simulink model "kay1024_freq_16ch_test"  (R2021b)
settings: Solver=VariableStepAuto  StartTime=0.0  StopTime=10.0  RelTol=1e-3
undefined symbols (not defined in the file): i
libraries: hdlBasic x1194, dspsrcs4 x16, vmcUtilities x1
(part 2 of 14)

== system kay1024_freq_16ch_test/Subsystem/Subsystem16/Subsystem7 ==
  In1 : Inport
  In2 : Inport  Port=2
  In3 : Inport  Port=3
  In4 : Inport  Port=4
  CORDIC ATAN : Subsystem  mask(Xilinx CORDIC ATAN){stages=15, pe_nbits=30, pe_binpt=18, pipeline_x=ones(1,15), prev_stages=15, pipeline=[1  1  1  1  1  1  1  1  1  1  1  1  1  1  1]}
      mask prompts: stages "Number of Processing Elements (integer value starting from 1)"; pe_nbits "X, Y Data Width"; pe_binpt "X, Y Binary Point Position"; pipeline_x "Latency for each Processing Element [1 0 0 1]"; prev_stages "Previous Number of Stages"; pipeline "Previous Pipeline Values"
      mask help: A parallel implementation, circular vectoring mode CORDIC processor for performing rectangular-to-polar conversion. The number of iteration stages (and resultant output accuracy) and the processor arithmetic precision are controlled by the mask customization.
      mask init: same as kay1024_freq_16ch_test/Subsystem/Subsystem16/Subsystem/CORDIC ATAN
      settings: CopyFcn=set_param(gcb, 'MaskSelfModifiable', 'on', 'LinkStatus', 'none');
      mask Help: eval('');xlDoc('-book','sysgen','-topic','CORDIC_ATAN');
      mask Display:
      | patch([0 iWidth iWidth 0],[0 0 iHeight iHeight] , bg);
      | patch(logoX,logoY , fg);
      | text(iCx-6,iCy,'z');
      | text(iCx,iCy+4,str);
      | port_label('input',1,'x');
      | port_label('input',2,'y');
      | port_label('output',1,'mag');
      | port_label('output',2,'atan');
      | plot([0 0 iWidth iWidth 0], [0 iHeight iHeight 0 0]);
  im0*im1 : hdlBasic/Mult  precision=Full  arith_type="Signed  (2's comp)"  n_bits=16  bin_pt=14  quantization=Truncate  overflow=Wrap  en=off  latency=3  use_behavioral_HDL=off  opt=Speed  use_embedded=on  optimum_pipeline=off  pipeline=on  use_rpm=on  placement_style=Triangular  XmcBlockStatus=1  maskContainerNames=group1  block_type=mult  block_config=sysgen:Mult_config  block_width=598  block_height=876
  re0*im1 : hdlBasic/Mult  precision=Full  arith_type="Signed  (2's comp)"  n_bits=16  bin_pt=14  quantization=Truncate  overflow=Wrap  en=off  latency=3  use_behavioral_HDL=off  opt=Speed  use_embedded=on  optimum_pipeline=off  pipeline=on  use_rpm=on  placement_style=Triangular  XmcBlockStatus=1  maskContainerNames=group1  block_type=mult  block_config=sysgen:Mult_config  block_width=598  block_height=876
  re0*im1-re1*im0 : hdlBasic/AddSub  mode=Subtraction  use_carryin=off  use_carryout=off  en=off  latency=1  precision=Full  arith_type=Unsigned  n_bits=16  bin_pt=14  quantization=Truncate  overflow=Wrap  use_behavioral_HDL=off  hw_selection=Fabric  pipelined=off  XmcBlockStatus=1  maskContainerNames=tabcontainer1  block_type=addsub  block_config=sysgen:Addsub_config
  re0*re1 : hdlBasic/Mult  precision=Full  arith_type="Signed  (2's comp)"  n_bits=16  bin_pt=14  quantization=Truncate  overflow=Wrap  en=off  latency=3  use_behavioral_HDL=off  opt=Speed  use_embedded=on  optimum_pipeline=off  pipeline=on  use_rpm=on  placement_style=Triangular  XmcBlockStatus=1  maskContainerNames=group1  block_type=mult  block_config=sysgen:Mult_config  block_width=598  block_height=876
  re0*re1+im0*im1 : hdlBasic/AddSub  mode=Addition  use_carryin=off  use_carryout=off  en=off  latency=1  precision=Full  arith_type=Unsigned  n_bits=16  bin_pt=14  quantization=Truncate  overflow=Wrap  use_behavioral_HDL=off  hw_selection=Fabric  pipelined=off  XmcBlockStatus=1  maskContainerNames=tabcontainer1  block_type=addsub  block_config=sysgen:Addsub_config
  re1*im0 : hdlBasic/Mult  precision=Full  arith_type="Signed  (2's comp)"  n_bits=16  bin_pt=14  quantization=Truncate  overflow=Wrap  en=off  latency=3  use_behavioral_HDL=off  opt=Speed  use_embedded=on  optimum_pipeline=off  pipeline=on  use_rpm=on  placement_style=Triangular  XmcBlockStatus=1  maskContainerNames=group1  block_type=mult  block_config=sysgen:Mult_config  block_width=598  block_height=876
  Z : Outport
  wires:
  In3/1 -> re1*im0/2, im0*im1/1
  re0*im1-re1*im0/1 -> CORDIC ATAN/2(y)
  In2/1 -> re0*re1/2, re1*im0/1
  In4/1 -> re0*im1/2, im0*im1/2
  re0*im1/1 -> re0*im1-re1*im0/1
  In1/1 -> re0*im1/1, re0*re1/1
  re0*re1/1 -> re0*re1+im0*im1/1
  im0*im1/1 -> re0*re1+im0*im1/2
  re0*re1+im0*im1/1 -> CORDIC ATAN/1(x)
  re1*im0/1 -> re0*im1-re1*im0/2
  CORDIC ATAN/2(Z) -> Z/1

== system kay1024_freq_16ch_test/Subsystem/Subsystem16/Subsystem/CORDIC ATAN ==
  note: The CORDIC algorithm is implemented in 3 steps.
      |
      | Step 1: Coarse Angle Rotation.  The algorithm converges only for angles between -pi/2 and pi/2, so if x < zero, the input vector is reflected
      | to the 1st or 3rd quadrant by making the x-coordinate non-negative.
      |
      | Step 2: Fine Angle Rotation.  For rectangular-to-polar conversion, the resulting vector is rotated through progressively smaller angles, such that y goes
      | to zero. In the i-th stage, the angular rotation is by either +/- atan(1/2^i), depending on whether or not its input y is less than or greater than zero.
      |
      | Step 3: Angle Correction. If there was a reflection applied in Step 1, this step applies the appropriate angle correction by subtracting it from +/- pi.
  x : Inport
  y : Inport  Port=2
  CORDIC Pipe Balance : hdlBasic/Delay  rst=off  en=off  latency=sum(pipeline)  reg_retiming=off  XmcBlockStatus=1  maskContainerNames=group1  block_type=delay  block_config=sysgen:Delay_config
  CORDIC Pipe Balance1 : hdlBasic/Delay  rst=off  en=off  latency=sum(pipeline)+1  reg_retiming=off  XmcBlockStatus=1  maskContainerNames=group1  block_type=delay  block_config=sysgen:Delay_config
  CORDIC Pipe Balance2 : hdlBasic/Delay  rst=off  en=off  latency=1  reg_retiming=off  XmcBlockStatus=1  maskContainerNames=group1  block_type=delay  block_config=sysgen:Delay_config
  CORDIC Fine Angle PE : Subsystem  mask(CORDIC parallel PE){}
      mask init:
      | [bg,fg] = xlcmap('XBlock',0);
      | iPos = get_param(gcb,'Position');
      | iWidth=iPos(3)-iPos(1); iHeight=iPos(4)-iPos(2);
      | iCx=iWidth/2;
      | iCy=iHeight/2;
      | [logoX, logoY] = xlogo(iPos);
      mask Display:
      | patch([0 iWidth iWidth 0],[0 0 iHeight iHeight] , bg);
      | patch(logoX,logoY , fg);
      | port_label('input',1,'x');
      | port_label('input',2,'y');
      | port_label('input',3,'z');
      | port_label('output',1,'X');
      | port_label('output',2,'Z');
      | plot([0 0 iWidth iWidth 0], [0 iHeight iHeight 0 0]);
  Constant : hdlBasic/Constant  const=0  gui_display_data_type=Fixed-point  arith_type=Signed (2's comp)  n_bits=pe_nbits  bin_pt=pe_binpt  preci_type=Single  exp_width=8  frac_width=24  explicit_period=off  period=1  XmcBlockStatus=1  maskContainerNames=tabcontainer1  block_type=constant  block_config=sysgen:Constant_config
  Quadrant Correct : Subsystem
      mask init:
      | [bg,fg] = xlcmap('XBlock',0);
      | iPos = get_param(gcb,'Position');
      | iWidth=iPos(3)-iPos(1); iHeight=iPos(4)-iPos(2);
      | iCx=iWidth/2;
      | iCy=iHeight/2;
      | [logoX, logoY] = xlogo(iPos);
      mask Display:
      | patch([0 iWidth iWidth 0],[0 0 iHeight iHeight] , bg);
      | patch(logoX,logoY , fg);
      | port_label('input',1,'Z in');
      | port_label('input',2,'sgn(y)');
      | port_label('input',3,'sgn(x)');
      | port_label('output',1,'Z');
      | plot([0 0 iWidth iWidth 0], [0 iHeight iHeight 0 0]);
  Quadrant Map : Subsystem
      mask init:
      | [bg,fg] = xlcmap('XBlock',0);
      | iPos = get_param(gcb,'Position');
      | iWidth=iPos(3)-iPos(1); iHeight=iPos(4)-iPos(2);
      | iCx=iWidth/2;
      | iCy=iHeight/2;
      | [logoX, logoY] = xlogo(iPos);
      mask Display:
      | patch([0 iWidth iWidth 0],[0 0 iHeight iHeight] , bg);
      | patch(logoX,logoY , fg);
      | port_label('input',1,'x');
      | port_label('input',2,'y');
      | port_label('output',1,'X');
      | port_label('output',2,'Y');
      | port_label('output',3,'sgn(y)');
      | port_label('output',4,'sgn(x)');
      | plot([0 0 iWidth iWidth 0], [0 iHeight iHeight 0 0]);
  X : Outport
  Z : Outport  Port=2
  wires:
  CORDIC Pipe Balance2/1 -> X/1
  CORDIC Fine Angle PE/1(X) -> CORDIC Pipe Balance2/1
  Quadrant Correct/1(Z) -> Z/1
  CORDIC Fine Angle PE/2(Z) -> Quadrant Correct/1(Z IN)
  CORDIC Pipe Balance1/1 -> Quadrant Correct/3(Z MUX SEL)
  CORDIC Pipe Balance/1 -> Quadrant Correct/2(PI_ addsub)
  Quadrant Map/4(sign(x)) -> CORDIC Pipe Balance1/1
  Quadrant Map/3(sign(y)) -> CORDIC Pipe Balance/1
  y/1 -> Quadrant Map/2(y)
  x/1 -> Quadrant Map/1(x)
  Quadrant Map/2(Y) -> CORDIC Fine Angle PE/2(y)
  Quadrant Map/1(X) -> CORDIC Fine Angle PE/1(x)
  Constant/1 -> CORDIC Fine Angle PE/3(z)

== system kay1024_freq_16ch_test/Subsystem/Subsystem16/Subsystem1/CORDIC ATAN ==
  note: The CORDIC algorithm is implemented in 3 steps.
      |
      | Step 1: Coarse Angle Rotation.  The algorithm converges only for angles between -pi/2 and pi/2, so if x < zero, the input vector is reflected
      | to the 1st or 3rd quadrant by making the x-coordinate non-negative.
      |
      | Step 2: Fine Angle Rotation.  For rectangular-to-polar conversion, the resulting vector is rotated through progressively smaller angles, such that y goes
      | to zero. In the i-th stage, the angular rotation is by either +/- atan(1/2^i), depending on whether or not its input y is less than or greater than zero.
      |
      | Step 3: Angle Correction. If there was a reflection applied in Step 1, this step applies the appropriate angle correction by subtracting it from +/- pi.
  x : Inport
  y : Inport  Port=2
  CORDIC Pipe Balance : hdlBasic/Delay  rst=off  en=off  latency=sum(pipeline)  reg_retiming=off  XmcBlockStatus=1  maskContainerNames=group1  block_type=delay  block_config=sysgen:Delay_config
  CORDIC Pipe Balance1 : hdlBasic/Delay  rst=off  en=off  latency=sum(pipeline)+1  reg_retiming=off  XmcBlockStatus=1  maskContainerNames=group1  block_type=delay  block_config=sysgen:Delay_config
  CORDIC Pipe Balance2 : hdlBasic/Delay  rst=off  en=off  latency=1  reg_retiming=off  XmcBlockStatus=1  maskContainerNames=group1  block_type=delay  block_config=sysgen:Delay_config
  CORDIC Fine Angle PE : Subsystem  mask(CORDIC parallel PE){}
      mask init:
      | [bg,fg] = xlcmap('XBlock',0);
      | iPos = get_param(gcb,'Position');
      | iWidth=iPos(3)-iPos(1); iHeight=iPos(4)-iPos(2);
      | iCx=iWidth/2;
      | iCy=iHeight/2;
      | [logoX, logoY] = xlogo(iPos);
      mask Display:
      | patch([0 iWidth iWidth 0],[0 0 iHeight iHeight] , bg);
      | patch(logoX,logoY , fg);
      | port_label('input',1,'x');
      | port_label('input',2,'y');
      | port_label('input',3,'z');
      | port_label('output',1,'X');
      | port_label('output',2,'Z');
      | plot([0 0 iWidth iWidth 0], [0 iHeight iHeight 0 0]);
  Constant : hdlBasic/Constant  const=0  gui_display_data_type=Fixed-point  arith_type=Signed (2's comp)  n_bits=pe_nbits  bin_pt=pe_binpt  preci_type=Single  exp_width=8  frac_width=24  explicit_period=off  period=1  XmcBlockStatus=1  maskContainerNames=tabcontainer1  block_type=constant  block_config=sysgen:Constant_config
  Quadrant Correct : Subsystem
      mask init:
      | [bg,fg] = xlcmap('XBlock',0);
      | iPos = get_param(gcb,'Position');
      | iWidth=iPos(3)-iPos(1); iHeight=iPos(4)-iPos(2);
      | iCx=iWidth/2;
      | iCy=iHeight/2;
      | [logoX, logoY] = xlogo(iPos);
      mask Display:
      | patch([0 iWidth iWidth 0],[0 0 iHeight iHeight] , bg);
      | patch(logoX,logoY , fg);
      | port_label('input',1,'Z in');
      | port_label('input',2,'sgn(y)');
      | port_label('input',3,'sgn(x)');
      | port_label('output',1,'Z');
      | plot([0 0 iWidth iWidth 0], [0 iHeight iHeight 0 0]);
  Quadrant Map : Subsystem
      mask init:
      | [bg,fg] = xlcmap('XBlock',0);
      | iPos = get_param(gcb,'Position');
      | iWidth=iPos(3)-iPos(1); iHeight=iPos(4)-iPos(2);
      | iCx=iWidth/2;
      | iCy=iHeight/2;
      | [logoX, logoY] = xlogo(iPos);
      mask Display:
      | patch([0 iWidth iWidth 0],[0 0 iHeight iHeight] , bg);
      | patch(logoX,logoY , fg);
      | port_label('input',1,'x');
      | port_label('input',2,'y');
      | port_label('output',1,'X');
      | port_label('output',2,'Y');
      | port_label('output',3,'sgn(y)');
      | port_label('output',4,'sgn(x)');
      | plot([0 0 iWidth iWidth 0], [0 iHeight iHeight 0 0]);
  X : Outport
  Z : Outport  Port=2
  wires:
  CORDIC Pipe Balance2/1 -> X/1
  CORDIC Fine Angle PE/1(X) -> CORDIC Pipe Balance2/1
  Quadrant Correct/1(Z) -> Z/1
  CORDIC Fine Angle PE/2(Z) -> Quadrant Correct/1(Z IN)
  CORDIC Pipe Balance1/1 -> Quadrant Correct/3(Z MUX SEL)
  CORDIC Pipe Balance/1 -> Quadrant Correct/2(PI_ addsub)
  Quadrant Map/4(sign(x)) -> CORDIC Pipe Balance1/1
  Quadrant Map/3(sign(y)) -> CORDIC Pipe Balance/1
  y/1 -> Quadrant Map/2(y)
  x/1 -> Quadrant Map/1(x)
  Quadrant Map/2(Y) -> CORDIC Fine Angle PE/2(y)
  Quadrant Map/1(X) -> CORDIC Fine Angle PE/1(x)
  Constant/1 -> CORDIC Fine Angle PE/3(z)

== system kay1024_freq_16ch_test/Subsystem/Subsystem16/Subsystem2/CORDIC ATAN ==
  note: The CORDIC algorithm is implemented in 3 steps.
      |
      | Step 1: Coarse Angle Rotation.  The algorithm converges only for angles between -pi/2 and pi/2, so if x < zero, the input vector is reflected
      | to the 1st or 3rd quadrant by making the x-coordinate non-negative.
      |
      | Step 2: Fine Angle Rotation.  For rectangular-to-polar conversion, the resulting vector is rotated through progressively smaller angles, such that y goes
      | to zero. In the i-th stage, the angular rotation is by either +/- atan(1/2^i), depending on whether or not its input y is less than or greater than zero.
      |
      | Step 3: Angle Correction. If there was a reflection applied in Step 1, this step applies the appropriate angle correction by subtracting it from +/- pi.
  x : Inport
  y : Inport  Port=2
  CORDIC Pipe Balance : hdlBasic/Delay  rst=off  en=off  latency=sum(pipeline)  reg_retiming=off  XmcBlockStatus=1  maskContainerNames=group1  block_type=delay  block_config=sysgen:Delay_config
  CORDIC Pipe Balance1 : hdlBasic/Delay  rst=off  en=off  latency=sum(pipeline)+1  reg_retiming=off  XmcBlockStatus=1  maskContainerNames=group1  block_type=delay  block_config=sysgen:Delay_config
  CORDIC Pipe Balance2 : hdlBasic/Delay  rst=off  en=off  latency=1  reg_retiming=off  XmcBlockStatus=1  maskContainerNames=group1  block_type=delay  block_config=sysgen:Delay_config
  CORDIC Fine Angle PE : Subsystem  mask(CORDIC parallel PE){}
      mask init:
      | [bg,fg] = xlcmap('XBlock',0);
      | iPos = get_param(gcb,'Position');
      | iWidth=iPos(3)-iPos(1); iHeight=iPos(4)-iPos(2);
      | iCx=iWidth/2;
      | iCy=iHeight/2;
      | [logoX, logoY] = xlogo(iPos);
      mask Display:
      | patch([0 iWidth iWidth 0],[0 0 iHeight iHeight] , bg);
      | patch(logoX,logoY , fg);
      | port_label('input',1,'x');
      | port_label('input',2,'y');
      | port_label('input',3,'z');
      | port_label('output',1,'X');
      | port_label('output',2,'Z');
      | plot([0 0 iWidth iWidth 0], [0 iHeight iHeight 0 0]);
  Constant : hdlBasic/Constant  const=0  gui_display_data_type=Fixed-point  arith_type=Signed (2's comp)  n_bits=pe_nbits  bin_pt=pe_binpt  preci_type=Single  exp_width=8  frac_width=24  explicit_period=off  period=1  XmcBlockStatus=1  maskContainerNames=tabcontainer1  block_type=constant  block_config=sysgen:Constant_config
  Quadrant Correct : Subsystem
      mask init:
      | [bg,fg] = xlcmap('XBlock',0);
      | iPos = get_param(gcb,'Position');
      | iWidth=iPos(3)-iPos(1); iHeight=iPos(4)-iPos(2);
      | iCx=iWidth/2;
      | iCy=iHeight/2;
      | [logoX, logoY] = xlogo(iPos);
      mask Display:
      | patch([0 iWidth iWidth 0],[0 0 iHeight iHeight] , bg);
      | patch(logoX,logoY , fg);
      | port_label('input',1,'Z in');
      | port_label('input',2,'sgn(y)');
      | port_label('input',3,'sgn(x)');
      | port_label('output',1,'Z');
      | plot([0 0 iWidth iWidth 0], [0 iHeight iHeight 0 0]);
  Quadrant Map : Subsystem
      mask init:
      | [bg,fg] = xlcmap('XBlock',0);
      | iPos = get_param(gcb,'Position');
      | iWidth=iPos(3)-iPos(1); iHeight=iPos(4)-iPos(2);
      | iCx=iWidth/2;
      | iCy=iHeight/2;
      | [logoX, logoY] = xlogo(iPos);
      mask Display:
      | patch([0 iWidth iWidth 0],[0 0 iHeight iHeight] , bg);
      | patch(logoX,logoY , fg);
      | port_label('input',1,'x');
      | port_label('input',2,'y');
      | port_label('output',1,'X');
      | port_label('output',2,'Y');
      | port_label('output',3,'sgn(y)');
      | port_label('output',4,'sgn(x)');
      | plot([0 0 iWidth iWidth 0], [0 iHeight iHeight 0 0]);
  X : Outport
  Z : Outport  Port=2
  wires:
  CORDIC Pipe Balance2/1 -> X/1
  CORDIC Fine Angle PE/1(X) -> CORDIC Pipe Balance2/1
  Quadrant Correct/1(Z) -> Z/1
  CORDIC Fine Angle PE/2(Z) -> Quadrant Correct/1(Z IN)
  CORDIC Pipe Balance1/1 -> Quadrant Correct/3(Z MUX SEL)
  CORDIC Pipe Balance/1 -> Quadrant Correct/2(PI_ addsub)
  Quadrant Map/4(sign(x)) -> CORDIC Pipe Balance1/1
  Quadrant Map/3(sign(y)) -> CORDIC Pipe Balance/1
  y/1 -> Quadrant Map/2(y)
  x/1 -> Quadrant Map/1(x)
  Quadrant Map/2(Y) -> CORDIC Fine Angle PE/2(y)
  Quadrant Map/1(X) -> CORDIC Fine Angle PE/1(x)
  Constant/1 -> CORDIC Fine Angle PE/3(z)

== system kay1024_freq_16ch_test/Subsystem/Subsystem16/Subsystem3/CORDIC ATAN ==
  note: The CORDIC algorithm is implemented in 3 steps.
      |
      | Step 1: Coarse Angle Rotation.  The algorithm converges only for angles between -pi/2 and pi/2, so if x < zero, the input vector is reflected
      | to the 1st or 3rd quadrant by making the x-coordinate non-negative.
      |
      | Step 2: Fine Angle Rotation.  For rectangular-to-polar conversion, the resulting vector is rotated through progressively smaller angles, such that y goes
      | to zero. In the i-th stage, the angular rotation is by either +/- atan(1/2^i), depending on whether or not its input y is less than or greater than zero.
      |
      | Step 3: Angle Correction. If there was a reflection applied in Step 1, this step applies the appropriate angle correction by subtracting it from +/- pi.
  x : Inport
  y : Inport  Port=2
  CORDIC Pipe Balance : hdlBasic/Delay  rst=off  en=off  latency=sum(pipeline)  reg_retiming=off  XmcBlockStatus=1  maskContainerNames=group1  block_type=delay  block_config=sysgen:Delay_config
  CORDIC Pipe Balance1 : hdlBasic/Delay  rst=off  en=off  latency=sum(pipeline)+1  reg_retiming=off  XmcBlockStatus=1  maskContainerNames=group1  block_type=delay  block_config=sysgen:Delay_config
  CORDIC Pipe Balance2 : hdlBasic/Delay  rst=off  en=off  latency=1  reg_retiming=off  XmcBlockStatus=1  maskContainerNames=group1  block_type=delay  block_config=sysgen:Delay_config
  CORDIC Fine Angle PE : Subsystem  mask(CORDIC parallel PE){}
      mask init:
      | [bg,fg] = xlcmap('XBlock',0);
      | iPos = get_param(gcb,'Position');
      | iWidth=iPos(3)-iPos(1); iHeight=iPos(4)-iPos(2);
      | iCx=iWidth/2;
      | iCy=iHeight/2;
      | [logoX, logoY] = xlogo(iPos);
      mask Display:
      | patch([0 iWidth iWidth 0],[0 0 iHeight iHeight] , bg);
      | patch(logoX,logoY , fg);
      | port_label('input',1,'x');
      | port_label('input',2,'y');
      | port_label('input',3,'z');
      | port_label('output',1,'X');
      | port_label('output',2,'Z');
      | plot([0 0 iWidth iWidth 0], [0 iHeight iHeight 0 0]);
  Constant : hdlBasic/Constant  const=0  gui_display_data_type=Fixed-point  arith_type=Signed (2's comp)  n_bits=pe_nbits  bin_pt=pe_binpt  preci_type=Single  exp_width=8  frac_width=24  explicit_period=off  period=1  XmcBlockStatus=1  maskContainerNames=tabcontainer1  block_type=constant  block_config=sysgen:Constant_config
  Quadrant Correct : Subsystem
      mask init:
      | [bg,fg] = xlcmap('XBlock',0);
      | iPos = get_param(gcb,'Position');
      | iWidth=iPos(3)-iPos(1); iHeight=iPos(4)-iPos(2);
      | iCx=iWidth/2;
      | iCy=iHeight/2;
      | [logoX, logoY] = xlogo(iPos);
      mask Display:
      | patch([0 iWidth iWidth 0],[0 0 iHeight iHeight] , bg);
      | patch(logoX,logoY , fg);
      | port_label('input',1,'Z in');
      | port_label('input',2,'sgn(y)');
      | port_label('input',3,'sgn(x)');
      | port_label('output',1,'Z');
      | plot([0 0 iWidth iWidth 0], [0 iHeight iHeight 0 0]);
  Quadrant Map : Subsystem
      mask init:
      | [bg,fg] = xlcmap('XBlock',0);
      | iPos = get_param(gcb,'Position');
      | iWidth=iPos(3)-iPos(1); iHeight=iPos(4)-iPos(2);
      | iCx=iWidth/2;
      | iCy=iHeight/2;
      | [logoX, logoY] = xlogo(iPos);
      mask Display:
      | patch([0 iWidth iWidth 0],[0 0 iHeight iHeight] , bg);
      | patch(logoX,logoY , fg);
      | port_label('input',1,'x');
      | port_label('input',2,'y');
      | port_label('output',1,'X');
      | port_label('output',2,'Y');
      | port_label('output',3,'sgn(y)');
      | port_label('output',4,'sgn(x)');
      | plot([0 0 iWidth iWidth 0], [0 iHeight iHeight 0 0]);
  X : Outport
  Z : Outport  Port=2
  wires:
  CORDIC Pipe Balance2/1 -> X/1
  CORDIC Fine Angle PE/1(X) -> CORDIC Pipe Balance2/1
  Quadrant Correct/1(Z) -> Z/1
  CORDIC Fine Angle PE/2(Z) -> Quadrant Correct/1(Z IN)
  CORDIC Pipe Balance1/1 -> Quadrant Correct/3(Z MUX SEL)
  CORDIC Pipe Balance/1 -> Quadrant Correct/2(PI_ addsub)
  Quadrant Map/4(sign(x)) -> CORDIC Pipe Balance1/1
  Quadrant Map/3(sign(y)) -> CORDIC Pipe Balance/1
  y/1 -> Quadrant Map/2(y)
  x/1 -> Quadrant Map/1(x)
  Quadrant Map/2(Y) -> CORDIC Fine Angle PE/2(y)
  Quadrant Map/1(X) -> CORDIC Fine Angle PE/1(x)
  Constant/1 -> CORDIC Fine Angle PE/3(z)

== system kay1024_freq_16ch_test/Subsystem/Subsystem16/Subsystem4/CORDIC ATAN ==
  note: The CORDIC algorithm is implemented in 3 steps.
      |
      | Step 1: Coarse Angle Rotation.  The algorithm converges only for angles between -pi/2 and pi/2, so if x < zero, the input vector is reflected
      | to the 1st or 3rd quadrant by making the x-coordinate non-negative.
      |
      | Step 2: Fine Angle Rotation.  For rectangular-to-polar conversion, the resulting vector is rotated through progressively smaller angles, such that y goes
      | to zero. In the i-th stage, the angular rotation is by either +/- atan(1/2^i), depending on whether or not its input y is less than or greater than zero.
      |
      | Step 3: Angle Correction. If there was a reflection applied in Step 1, this step applies the appropriate angle correction by subtracting it from +/- pi.
  x : Inport
  y : Inport  Port=2
  CORDIC Pipe Balance : hdlBasic/Delay  rst=off  en=off  latency=sum(pipeline)  reg_retiming=off  XmcBlockStatus=1  maskContainerNames=group1  block_type=delay  block_config=sysgen:Delay_config
  CORDIC Pipe Balance1 : hdlBasic/Delay  rst=off  en=off  latency=sum(pipeline)+1  reg_retiming=off  XmcBlockStatus=1  maskContainerNames=group1  block_type=delay  block_config=sysgen:Delay_config
  CORDIC Pipe Balance2 : hdlBasic/Delay  rst=off  en=off  latency=1  reg_retiming=off  XmcBlockStatus=1  maskContainerNames=group1  block_type=delay  block_config=sysgen:Delay_config
  CORDIC Fine Angle PE : Subsystem  mask(CORDIC parallel PE){}
      mask init:
      | [bg,fg] = xlcmap('XBlock',0);
      | iPos = get_param(gcb,'Position');
      | iWidth=iPos(3)-iPos(1); iHeight=iPos(4)-iPos(2);
      | iCx=iWidth/2;
      | iCy=iHeight/2;
      | [logoX, logoY] = xlogo(iPos);
      mask Display:
      | patch([0 iWidth iWidth 0],[0 0 iHeight iHeight] , bg);
      | patch(logoX,logoY , fg);
      | port_label('input',1,'x');
      | port_label('input',2,'y');
      | port_label('input',3,'z');
      | port_label('output',1,'X');
      | port_label('output',2,'Z');
      | plot([0 0 iWidth iWidth 0], [0 iHeight iHeight 0 0]);
  Constant : hdlBasic/Constant  const=0  gui_display_data_type=Fixed-point  arith_type=Signed (2's comp)  n_bits=pe_nbits  bin_pt=pe_binpt  preci_type=Single  exp_width=8  frac_width=24  explicit_period=off  period=1  XmcBlockStatus=1  maskContainerNames=tabcontainer1  block_type=constant  block_config=sysgen:Constant_config
  Quadrant Correct : Subsystem
      mask init:
      | [bg,fg] = xlcmap('XBlock',0);
      | iPos = get_param(gcb,'Position');
      | iWidth=iPos(3)-iPos(1); iHeight=iPos(4)-iPos(2);
      | iCx=iWidth/2;
      | iCy=iHeight/2;
      | [logoX, logoY] = xlogo(iPos);
      mask Display:
      | patch([0 iWidth iWidth 0],[0 0 iHeight iHeight] , bg);
      | patch(logoX,logoY , fg);
      | port_label('input',1,'Z in');
      | port_label('input',2,'sgn(y)');
      | port_label('input',3,'sgn(x)');
      | port_label('output',1,'Z');
      | plot([0 0 iWidth iWidth 0], [0 iHeight iHeight 0 0]);
  Quadrant Map : Subsystem
      mask init:
      | [bg,fg] = xlcmap('XBlock',0);
      | iPos = get_param(gcb,'Position');
      | iWidth=iPos(3)-iPos(1); iHeight=iPos(4)-iPos(2);
      | iCx=iWidth/2;
      | iCy=iHeight/2;
      | [logoX, logoY] = xlogo(iPos);
      mask Display:
      | patch([0 iWidth iWidth 0],[0 0 iHeight iHeight] , bg);
      | patch(logoX,logoY , fg);
      | port_label('input',1,'x');
      | port_label('input',2,'y');
      | port_label('output',1,'X');
      | port_label('output',2,'Y');
      | port_label('output',3,'sgn(y)');
      | port_label('output',4,'sgn(x)');
      | plot([0 0 iWidth iWidth 0], [0 iHeight iHeight 0 0]);
  X : Outport
  Z : Outport  Port=2
  wires:
  CORDIC Pipe Balance2/1 -> X/1
  CORDIC Fine Angle PE/1(X) -> CORDIC Pipe Balance2/1
  Quadrant Correct/1(Z) -> Z/1
  CORDIC Fine Angle PE/2(Z) -> Quadrant Correct/1(Z IN)
  CORDIC Pipe Balance1/1 -> Quadrant Correct/3(Z MUX SEL)
  CORDIC Pipe Balance/1 -> Quadrant Correct/2(PI_ addsub)
  Quadrant Map/4(sign(x)) -> CORDIC Pipe Balance1/1
  Quadrant Map/3(sign(y)) -> CORDIC Pipe Balance/1
  y/1 -> Quadrant Map/2(y)
  x/1 -> Quadrant Map/1(x)
  Quadrant Map/2(Y) -> CORDIC Fine Angle PE/2(y)
  Quadrant Map/1(X) -> CORDIC Fine Angle PE/1(x)
  Constant/1 -> CORDIC Fine Angle PE/3(z)

== system kay1024_freq_16ch_test/Subsystem/Subsystem16/Subsystem5/CORDIC ATAN ==
  note: The CORDIC algorithm is implemented in 3 steps.
      |
      | Step 1: Coarse Angle Rotation.  The algorithm converges only for angles between -pi/2 and pi/2, so if x < zero, the input vector is reflected
      | to the 1st or 3rd quadrant by making the x-coordinate non-negative.
      |
      | Step 2: Fine Angle Rotation.  For rectangular-to-polar conversion, the resulting vector is rotated through progressively smaller angles, such that y goes
      | to zero. In the i-th stage, the angular rotation is by either +/- atan(1/2^i), depending on whether or not its input y is less than or greater than zero.
      |
      | Step 3: Angle Correction. If there was a reflection applied in Step 1, this step applies the appropriate angle correction by subtracting it from +/- pi.
  x : Inport
  y : Inport  Port=2
  CORDIC Pipe Balance : hdlBasic/Delay  rst=off  en=off  latency=sum(pipeline)  reg_retiming=off  XmcBlockStatus=1  maskContainerNames=group1  block_type=delay  block_config=sysgen:Delay_config
  CORDIC Pipe Balance1 : hdlBasic/Delay  rst=off  en=off  latency=sum(pipeline)+1  reg_retiming=off  XmcBlockStatus=1  maskContainerNames=group1  block_type=delay  block_config=sysgen:Delay_config
  CORDIC Pipe Balance2 : hdlBasic/Delay  rst=off  en=off  latency=1  reg_retiming=off  XmcBlockStatus=1  maskContainerNames=group1  block_type=delay  block_config=sysgen:Delay_config
  CORDIC Fine Angle PE : Subsystem  mask(CORDIC parallel PE){}
      mask init:
      | [bg,fg] = xlcmap('XBlock',0);
      | iPos = get_param(gcb,'Position');
      | iWidth=iPos(3)-iPos(1); iHeight=iPos(4)-iPos(2);
      | iCx=iWidth/2;
      | iCy=iHeight/2;
      | [logoX, logoY] = xlogo(iPos);
      mask Display:
      | patch([0 iWidth iWidth 0],[0 0 iHeight iHeight] , bg);
      | patch(logoX,logoY , fg);
      | port_label('input',1,'x');
      | port_label('input',2,'y');
      | port_label('input',3,'z');
      | port_label('output',1,'X');
      | port_label('output',2,'Z');
      | plot([0 0 iWidth iWidth 0], [0 iHeight iHeight 0 0]);
  Constant : hdlBasic/Constant  const=0  gui_display_data_type=Fixed-point  arith_type=Signed (2's comp)  n_bits=pe_nbits  bin_pt=pe_binpt  preci_type=Single  exp_width=8  frac_width=24  explicit_period=off  period=1  XmcBlockStatus=1  maskContainerNames=tabcontainer1  block_type=constant  block_config=sysgen:Constant_config
  Quadrant Correct : Subsystem
      mask init:
      | [bg,fg] = xlcmap('XBlock',0);
      | iPos = get_param(gcb,'Position');
      | iWidth=iPos(3)-iPos(1); iHeight=iPos(4)-iPos(2);
      | iCx=iWidth/2;
      | iCy=iHeight/2;
      | [logoX, logoY] = xlogo(iPos);
      mask Display:
      | patch([0 iWidth iWidth 0],[0 0 iHeight iHeight] , bg);
      | patch(logoX,logoY , fg);
      | port_label('input',1,'Z in');
      | port_label('input',2,'sgn(y)');
      | port_label('input',3,'sgn(x)');
      | port_label('output',1,'Z');
      | plot([0 0 iWidth iWidth 0], [0 iHeight iHeight 0 0]);
  Quadrant Map : Subsystem
      mask init:
      | [bg,fg] = xlcmap('XBlock',0);
      | iPos = get_param(gcb,'Position');
      | iWidth=iPos(3)-iPos(1); iHeight=iPos(4)-iPos(2);
      | iCx=iWidth/2;
      | iCy=iHeight/2;
      | [logoX, logoY] = xlogo(iPos);
      mask Display:
      | patch([0 iWidth iWidth 0],[0 0 iHeight iHeight] , bg);
      | patch(logoX,logoY , fg);
      | port_label('input',1,'x');
      | port_label('input',2,'y');
      | port_label('output',1,'X');
      | port_label('output',2,'Y');
      | port_label('output',3,'sgn(y)');
      | port_label('output',4,'sgn(x)');
      | plot([0 0 iWidth iWidth 0], [0 iHeight iHeight 0 0]);
  X : Outport
  Z : Outport  Port=2
  wires:
  CORDIC Pipe Balance2/1 -> X/1
  CORDIC Fine Angle PE/1(X) -> CORDIC Pipe Balance2/1
  Quadrant Correct/1(Z) -> Z/1
  CORDIC Fine Angle PE/2(Z) -> Quadrant Correct/1(Z IN)
  CORDIC Pipe Balance1/1 -> Quadrant Correct/3(Z MUX SEL)
  CORDIC Pipe Balance/1 -> Quadrant Correct/2(PI_ addsub)
  Quadrant Map/4(sign(x)) -> CORDIC Pipe Balance1/1
  Quadrant Map/3(sign(y)) -> CORDIC Pipe Balance/1
  y/1 -> Quadrant Map/2(y)
  x/1 -> Quadrant Map/1(x)
  Quadrant Map/2(Y) -> CORDIC Fine Angle PE/2(y)
  Quadrant Map/1(X) -> CORDIC Fine Angle PE/1(x)
  Constant/1 -> CORDIC Fine Angle PE/3(z)

== system kay1024_freq_16ch_test/Subsystem/Subsystem16/Subsystem6/CORDIC ATAN ==
  note: The CORDIC algorithm is implemented in 3 steps.
      |
      | Step 1: Coarse Angle Rotation.  The algorithm converges only for angles between -pi/2 and pi/2, so if x < zero, the input vector is reflected
      | to the 1st or 3rd quadrant by making the x-coordinate non-negative.
      |
      | Step 2: Fine Angle Rotation.  For rectangular-to-polar conversion, the resulting vector is rotated through progressively smaller angles, such that y goes
      | to zero. In the i-th stage, the angular rotation is by either +/- atan(1/2^i), depending on whether or not its input y is less than or greater than zero.
      |
      | Step 3: Angle Correction. If there was a reflection applied in Step 1, this step applies the appropriate angle correction by subtracting it from +/- pi.
  x : Inport
  y : Inport  Port=2
  CORDIC Pipe Balance : hdlBasic/Delay  rst=off  en=off  latency=sum(pipeline)  reg_retiming=off  XmcBlockStatus=1  maskContainerNames=group1  block_type=delay  block_config=sysgen:Delay_config
  CORDIC Pipe Balance1 : hdlBasic/Delay  rst=off  en=off  latency=sum(pipeline)+1  reg_retiming=off  XmcBlockStatus=1  maskContainerNames=group1  block_type=delay  block_config=sysgen:Delay_config
  CORDIC Pipe Balance2 : hdlBasic/Delay  rst=off  en=off  latency=1  reg_retiming=off  XmcBlockStatus=1  maskContainerNames=group1  block_type=delay  block_config=sysgen:Delay_config
  CORDIC Fine Angle PE : Subsystem  mask(CORDIC parallel PE){}
      mask init:
      | [bg,fg] = xlcmap('XBlock',0);
      | iPos = get_param(gcb,'Position');
      | iWidth=iPos(3)-iPos(1); iHeight=iPos(4)-iPos(2);
      | iCx=iWidth/2;
      | iCy=iHeight/2;
      | [logoX, logoY] = xlogo(iPos);
      mask Display:
      | patch([0 iWidth iWidth 0],[0 0 iHeight iHeight] , bg);
      | patch(logoX,logoY , fg);
      | port_label('input',1,'x');
      | port_label('input',2,'y');
      | port_label('input',3,'z');
      | port_label('output',1,'X');
      | port_label('output',2,'Z');
      | plot([0 0 iWidth iWidth 0], [0 iHeight iHeight 0 0]);
  Constant : hdlBasic/Constant  const=0  gui_display_data_type=Fixed-point  arith_type=Signed (2's comp)  n_bits=pe_nbits  bin_pt=pe_binpt  preci_type=Single  exp_width=8  frac_width=24  explicit_period=off  period=1  XmcBlockStatus=1  maskContainerNames=tabcontainer1  block_type=constant  block_config=sysgen:Constant_config
  Quadrant Correct : Subsystem
      mask init:
      | [bg,fg] = xlcmap('XBlock',0);
      | iPos = get_param(gcb,'Position');
      | iWidth=iPos(3)-iPos(1); iHeight=iPos(4)-iPos(2);
      | iCx=iWidth/2;
      | iCy=iHeight/2;
      | [logoX, logoY] = xlogo(iPos);
      mask Display:
      | patch([0 iWidth iWidth 0],[0 0 iHeight iHeight] , bg);
      | patch(logoX,logoY , fg);
      | port_label('input',1,'Z in');
      | port_label('input',2,'sgn(y)');
      | port_label('input',3,'sgn(x)');
      | port_label('output',1,'Z');
      | plot([0 0 iWidth iWidth 0], [0 iHeight iHeight 0 0]);
  Quadrant Map : Subsystem
      mask init:
      | [bg,fg] = xlcmap('XBlock',0);
      | iPos = get_param(gcb,'Position');
      | iWidth=iPos(3)-iPos(1); iHeight=iPos(4)-iPos(2);
      | iCx=iWidth/2;
      | iCy=iHeight/2;
      | [logoX, logoY] = xlogo(iPos);
      mask Display:
      | patch([0 iWidth iWidth 0],[0 0 iHeight iHeight] , bg);
      | patch(logoX,logoY , fg);
      | port_label('input',1,'x');
      | port_label('input',2,'y');
      | port_label('output',1,'X');
      | port_label('output',2,'Y');
      | port_label('output',3,'sgn(y)');
      | port_label('output',4,'sgn(x)');
      | plot([0 0 iWidth iWidth 0], [0 iHeight iHeight 0 0]);
  X : Outport
  Z : Outport  Port=2
  wires:
  CORDIC Pipe Balance2/1 -> X/1
  CORDIC Fine Angle PE/1(X) -> CORDIC Pipe Balance2/1
  Quadrant Correct/1(Z) -> Z/1
  CORDIC Fine Angle PE/2(Z) -> Quadrant Correct/1(Z IN)
  CORDIC Pipe Balance1/1 -> Quadrant Correct/3(Z MUX SEL)
  CORDIC Pipe Balance/1 -> Quadrant Correct/2(PI_ addsub)
  Quadrant Map/4(sign(x)) -> CORDIC Pipe Balance1/1
  Quadrant Map/3(sign(y)) -> CORDIC Pipe Balance/1
  y/1 -> Quadrant Map/2(y)
  x/1 -> Quadrant Map/1(x)
  Quadrant Map/2(Y) -> CORDIC Fine Angle PE/2(y)
  Quadrant Map/1(X) -> CORDIC Fine Angle PE/1(x)
  Constant/1 -> CORDIC Fine Angle PE/3(z)

== system kay1024_freq_16ch_test/Subsystem/Subsystem16/Subsystem7/CORDIC ATAN ==
  note: The CORDIC algorithm is implemented in 3 steps.
      |
      | Step 1: Coarse Angle Rotation.  The algorithm converges only for angles between -pi/2 and pi/2, so if x < zero, the input vector is reflected
      | to the 1st or 3rd quadrant by making the x-coordinate non-negative.
      |
      | Step 2: Fine Angle Rotation.  For rectangular-to-polar conversion, the resulting vector is rotated through progressively smaller angles, such that y goes
      | to zero. In the i-th stage, the angular rotation is by either +/- atan(1/2^i), depending on whether or not its input y is less than or greater than zero.
      |
      | Step 3: Angle Correction. If there was a reflection applied in Step 1, this step applies the appropriate angle correction by subtracting it from +/- pi.
  x : Inport
  y : Inport  Port=2
  CORDIC Pipe Balance : hdlBasic/Delay  rst=off  en=off  latency=sum(pipeline)  reg_retiming=off  XmcBlockStatus=1  maskContainerNames=group1  block_type=delay  block_config=sysgen:Delay_config
  CORDIC Pipe Balance1 : hdlBasic/Delay  rst=off  en=off  latency=sum(pipeline)+1  reg_retiming=off  XmcBlockStatus=1  maskContainerNames=group1  block_type=delay  block_config=sysgen:Delay_config
  CORDIC Pipe Balance2 : hdlBasic/Delay  rst=off  en=off  latency=1  reg_retiming=off  XmcBlockStatus=1  maskContainerNames=group1  block_type=delay  block_config=sysgen:Delay_config
  CORDIC Fine Angle PE : Subsystem  mask(CORDIC parallel PE){}
      mask init:
      | [bg,fg] = xlcmap('XBlock',0);
      | iPos = get_param(gcb,'Position');
      | iWidth=iPos(3)-iPos(1); iHeight=iPos(4)-iPos(2);
      | iCx=iWidth/2;
      | iCy=iHeight/2;
      | [logoX, logoY] = xlogo(iPos);
      mask Display:
      | patch([0 iWidth iWidth 0],[0 0 iHeight iHeight] , bg);
      | patch(logoX,logoY , fg);
      | port_label('input',1,'x');
      | port_label('input',2,'y');
      | port_label('input',3,'z');
      | port_label('output',1,'X');
      | port_label('output',2,'Z');
      | plot([0 0 iWidth iWidth 0], [0 iHeight iHeight 0 0]);
  Constant : hdlBasic/Constant  const=0  gui_display_data_type=Fixed-point  arith_type=Signed (2's comp)  n_bits=pe_nbits  bin_pt=pe_binpt  preci_type=Single  exp_width=8  frac_width=24  explicit_period=off  period=1  XmcBlockStatus=1  maskContainerNames=tabcontainer1  block_type=constant  block_config=sysgen:Constant_config
  Quadrant Correct : Subsystem
      mask init:
      | [bg,fg] = xlcmap('XBlock',0);
      | iPos = get_param(gcb,'Position');
      | iWidth=iPos(3)-iPos(1); iHeight=iPos(4)-iPos(2);
      | iCx=iWidth/2;
      | iCy=iHeight/2;
      | [logoX, logoY] = xlogo(iPos);
      mask Display:
      | patch([0 iWidth iWidth 0],[0 0 iHeight iHeight] , bg);
      | patch(logoX,logoY , fg);
      | port_label('input',1,'Z in');
      | port_label('input',2,'sgn(y)');
      | port_label('input',3,'sgn(x)');
      | port_label('output',1,'Z');
      | plot([0 0 iWidth iWidth 0], [0 iHeight iHeight 0 0]);
  Quadrant Map : Subsystem
      mask init:
      | [bg,fg] = xlcmap('XBlock',0);
      | iPos = get_param(gcb,'Position');
      | iWidth=iPos(3)-iPos(1); iHeight=iPos(4)-iPos(2);
      | iCx=iWidth/2;
      | iCy=iHeight/2;
      | [logoX, logoY] = xlogo(iPos);
      mask Display:
      | patch([0 iWidth iWidth 0],[0 0 iHeight iHeight] , bg);
      | patch(logoX,logoY , fg);
      | port_label('input',1,'x');
      | port_label('input',2,'y');
      | port_label('output',1,'X');
      | port_label('output',2,'Y');
      | port_label('output',3,'sgn(y)');
      | port_label('output',4,'sgn(x)');
      | plot([0 0 iWidth iWidth 0], [0 iHeight iHeight 0 0]);
  X : Outport
  Z : Outport  Port=2
  wires:
  CORDIC Pipe Balance2/1 -> X/1
  CORDIC Fine Angle PE/1(X) -> CORDIC Pipe Balance2/1
  Quadrant Correct/1(Z) -> Z/1
  CORDIC Fine Angle PE/2(Z) -> Quadrant Correct/1(Z IN)
  CORDIC Pipe Balance1/1 -> Quadrant Correct/3(Z MUX SEL)
  CORDIC Pipe Balance/1 -> Quadrant Correct/2(PI_ addsub)
  Quadrant Map/4(sign(x)) -> CORDIC Pipe Balance1/1
  Quadrant Map/3(sign(y)) -> CORDIC Pipe Balance/1
  y/1 -> Quadrant Map/2(y)
  x/1 -> Quadrant Map/1(x)
  Quadrant Map/2(Y) -> CORDIC Fine Angle PE/2(y)
  Quadrant Map/1(X) -> CORDIC Fine Angle PE/1(x)
  Constant/1 -> CORDIC Fine Angle PE/3(z)
